simulink model "Prueba_kernel_pwm"  (R2025a)
settings: Solver=FixedStepDiscrete  StartTime=0.0  StopTime=1000  FixedStep=0.01  RelTol=1e-3
undefined symbols (not defined in the file or in its folder): Serial_Port, Standard_Devices
libraries: sldrtlib x1
settings Model: SimulationMode=external  Creator=aldo_  LastModifiedBy=aldo_
settings HardwareCC: ProdBitPerLong=64.0  ProdHWDeviceType=Intel->x86-64 (Linux 64)
settings RTWCC: SystemTargetFile=sldrt.tlc  TemplateMakefile=sldrt.tmf  RTWCompilerOptimization=on  Description=Simulink Desktop Real-Time
settings CodeAppCC: MaxIdLength=95.0
settings SimulinkDesktopRealTimeCC: ExtModeTransport=0.0  ExtModeStaticAllocSize=1000000.0  TargetLibSuffix=_sldrt.a  TargetPreCompLibLocation=C:\Program Files\MATLAB\R2025a\toolbox\sldrt\lib\win64  MultiwordLength=2048.0  DynamicStringBufferSize=256.0  ParMdlRefBuildCompliant=on  PreserveMATLABNamespacesInGeneratedCode=on  SubcomponentCodeInterfacePackaging=Reusable function

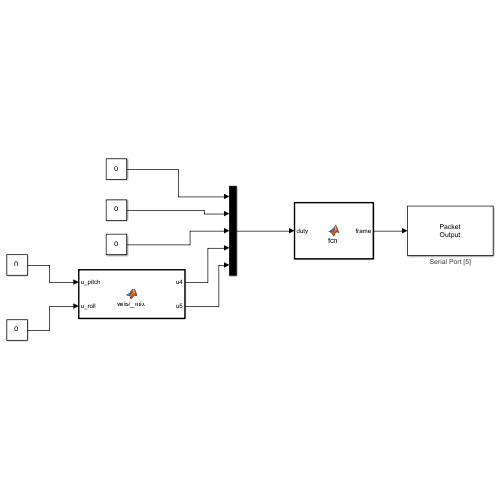
[thumbnail: Simulink's stored preview of the top-level diagram]
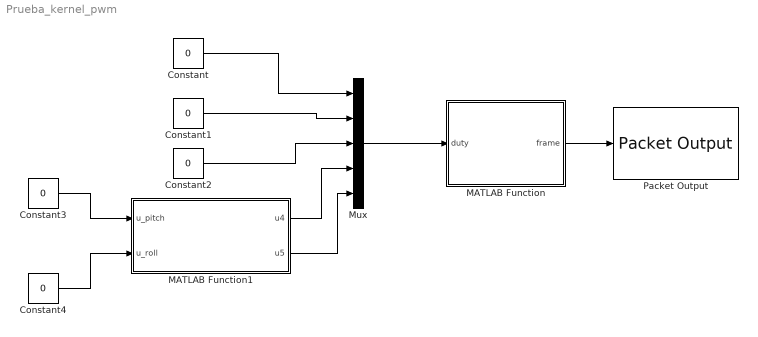
== system Prueba_kernel_pwm ==
  Constant{,1..4} (5 alike) : Constant  Value=0
  MATLAB Function : MATLAB Function  TreatAsAtomicUnit=on
  MATLAB Function1 : MATLAB Function  TreatAsAtomicUnit=on
  Mux : Mux  Inputs=5
  Packet Output : sldrtlib/Packet Output  SampleTime=0.01  MaxMissedTicks=10  ShowMissedTicks=off  YieldWhenWaiting=off  DrvName=Standard_Devices/Serial_Port  DrvAddress=5  DrvOptions=[115200 8 0 0 0 0 0 0]  PacketSize=14  DataTypes='14*uint8'  ShowReady=off  ShowError=off  PacketID=1  ByteOrder=1  InitialValue=[]  FinalValue=[]
      settings: AttributesFormatString=Serial Port [5]
  wires:
  Constant/1 -> Mux/1
  Constant2/1 -> Mux/3
  Constant1/1 -> Mux/2
  Mux/1 -> MATLAB Function/1(duty)
  MATLAB Function/1(frame) -> Packet Output/1
  Constant3/1 -> MATLAB Function1/1(u_pitch)
  Constant4/1 -> MATLAB Function1/2(u_roll)
  MATLAB Function1/1(u4) -> Mux/4
  MATLAB Function1/2(u5) -> Mux/5

== matlab function Prueba_kernel_pwm/MATLAB Function ==
  data: duty input; frame output
function frame = fcn(duty)
  frame = armdroid_pwm_frame(duty);

== matlab function Prueba_kernel_pwm/MATLAB Function1 ==
  data: u_pitch input; u4 output; u_roll input; u5 output
function [u4, u5] = wrist_mix(u_pitch, u_roll)
%WRIST_MIX  Differential wrist: joint commands -> motor 4/5 commands.
%  Matches power-app firmware with MOTOR_DIR_SIGN_INIT M5 = -1.
%  Roll  only: M4 and M5 physically opposite (same as hand held 'I'/'J').
%  Pitch only: M4 and M5 physically in the same direction.
s5 = -1;                              % firmware inverts motor 5
u4 = u_pitch + u_roll;
u5 = s5 * (u_pitch - u_roll);
m  = max([1, abs(u4), abs(u5)]);      % keep the motion direction if > 1
u4 = u4 / m;
u5 = u5 / m;
